simulink library "tec_holder_lib"  (R2025b)
settings: Solver=VariableStepAuto  StartTime=0.0  StopTime=10.0  RelTol=1e-3
undefined symbols (not defined in the file or in its folder): u0
settings Model: Creator=wardenaar  LastModifiedBy=wardenaar

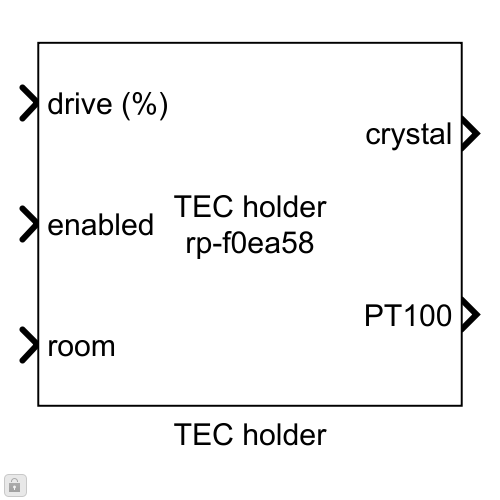
[thumbnail: Simulink's stored preview of the top-level diagram]
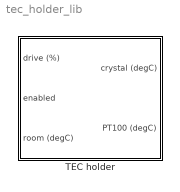
== system tec_holder_lib ==
  TEC holder : Subsystem  mask(TEC holder (rp-f0ea58)){a=0.495, b=0.00067, c=0.261, d=0.00044, kap=-0.0014, t1=312, t1_off=411, t2=12.2, theta=2.3, z=64.5, ta=80.1, tp=6.7, T0=22.2, Ta0=22.2}
      mask prompts: a "Heating map a (degC per %)"; b "Heating map b (degC per %^2)"; c "Cooling map c (degC per %)"; d "Cooling map d (degC per %^2)"; kap "Temperature term kap (1/degC)"; t1 "Slow pole, bridge enabled t1 (s)"; t1_off "Slow pole, bridge off t1_off (s)"; t2 "Crystal lag t2 (s)"; theta "Delay theta (s)"; z "PT100 lead z (s)"; ta "PT100 lag ta (s)"; tp "PT100 sensor lag tp (s)"; T0 "Initial crystal temperature T0 (degC)"; Ta0 "Room at the start Ta0 (degC)"
      mask help:
      | Thermal model of the QCM calibration holder on its Peltier, fitted on 14 Nov 2026 to an open-loop PRBS test on rp-f0ea58 (tools/README.md, section 9).
      |
      | Inputs: TEC drive in % (+ heats, limited to +-100), bridge enabled (0/1), room temperature (degC). Outputs: crystal and PT100 temperature (degC).
      |
      | Small signal around 40 degC: crystal = 0.47 e^(-2.3 s)/((320 s + 1)(12.2 s + 1)) per % drive; PT100 = crystal (64.5 s + 1)/((80.1 s + 1)(6.7 s + 1)).
      mask init:
      | % Drive that holds the crystal at T0 in a room at Ta0: the delay line starts with it.
      | dT = T0 - Ta0;
      | w = dT/(1 - kap*dT);
      | if w >= 0
      |     if b == 0, u0 = w/a; else, u0 = (a - sqrt(max(a^2 - 4*b*w, 0)))/(2*b); end
      | else
      |     if d == 0, u0 = w/c; else, u0 = (-c + sqrt(max(c^2 + 4*d*w, 0)))/(2*d); end
      | end
      | kz = z/ta;
      mask Display:
      | disp('TEC holder\nrp-f0ea58');
      | port_label('input', 1, 'drive (%)');
      | port_label('input', 2, 'enabled');
      | port_label('input', 3, 'room');
      | port_label('output', 1, 'crystal');
      | port_label('output', 2, 'PT100');

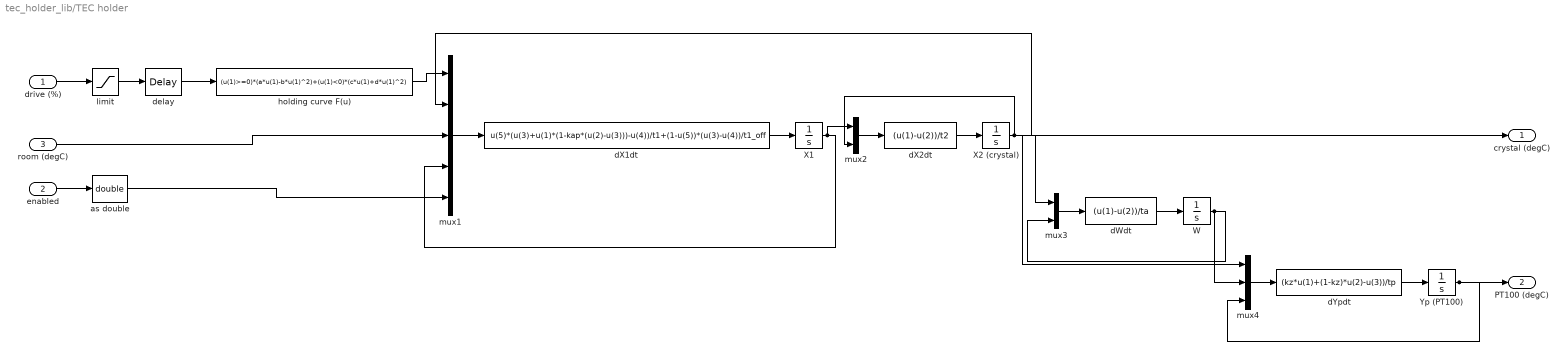
== system tec_holder_lib/TEC holder ==
  drive (%) : Inport
  enabled : Inport  Port=2
  room (degC) : Inport  Port=3
  W : Integrator  InitialCondition=T0
  X1 : Integrator  InitialCondition=T0
  X2 (crystal) : Integrator  InitialCondition=T0
  Yp (PT100) : Integrator  InitialCondition=T0
  as double : DataTypeConversion  OutDataTypeStr=double  SaturateOnIntegerOverflow=off  RndMeth=Floor
  dWdt : Fcn  Expr=(u(1)-u(2))/ta
  dX1dt : Fcn  Expr=u(5)*(u(3)+u(1)*(1-kap*(u(2)-u(3)))-u(4))/t1+(1-u(5))*(u(3)-u(4))/t1_off
  dX2dt : Fcn  Expr=(u(1)-u(2))/t2
  dYpdt : Fcn  Expr=(kz*u(1)+(1-kz)*u(2)-u(3))/tp
  delay : TransportDelay  DelayTime=theta  InitialOutput=u0
  holding curve F(u) : Fcn  Expr=(u(1)>=0)*(a*u(1)-b*u(1)^2)+(u(1)<0)*(c*u(1)+d*u(1)^2)
  limit : Saturate  UpperLimit=100  LowerLimit=-100
  mux1 : Mux  Inputs=5
  mux2 : Mux  Inputs=2
  mux3 : Mux  Inputs=2
  mux4 : Mux  Inputs=3
  crystal (degC) : Outport
  PT100 (degC) : Outport  Port=2
  wires:
  drive (%)/1 -> limit/1
  limit/1 -> delay/1
  delay/1 -> holding curve F(u)/1
  holding curve F(u)/1 -> mux1/1
  X2 (crystal)/1 -> mux1/2, mux2/2, mux3/1, mux4/1, crystal (degC)/1
  room (degC)/1 -> mux1/3
  X1/1 -> mux1/4, mux2/1
  enabled/1 -> as double/1
  as double/1 -> mux1/5
  mux1/1 -> dX1dt/1
  dX1dt/1 -> X1/1
  mux2/1 -> dX2dt/1
  dX2dt/1 -> X2 (crystal)/1
  W/1 -> mux3/2, mux4/2
  mux3/1 -> dWdt/1
  dWdt/1 -> W/1
  Yp (PT100)/1 -> mux4/3, PT100 (degC)/1
  mux4/1 -> dYpdt/1
  dYpdt/1 -> Yp (PT100)/1
